simulink model "Histogram_equization_simulink"  (R2023b)
settings: Solver=VariableStepAuto  StartTime=0.0  StopTime=10.0  RelTol=1e-3
libraries: visionanalysis x1, visionsources x1
settings Model: Creator=snmz4  LastModifiedBy=snmz4

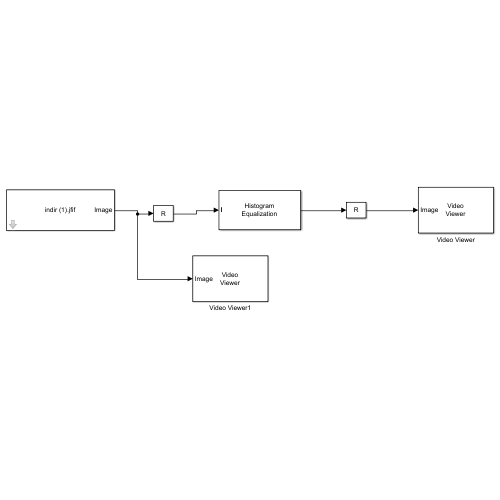
[thumbnail: Simulink's stored preview of the top-level diagram]
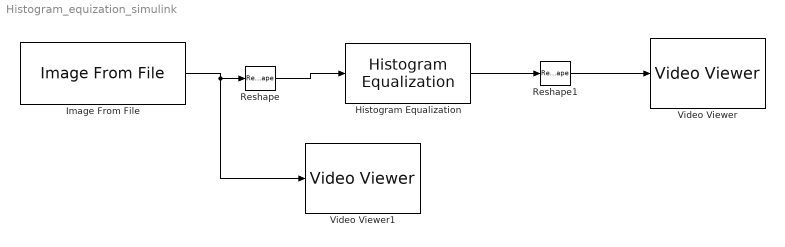
== system Histogram_equization_simulink ==
  Histogram Equalization : visionanalysis/Histogram Equalization  specify=Uniform  numbins=64  src=Specify via dialog  hist=ones(1,64)
  Image From File : visionsources/Image From File  Tag=vipblks_nd  FileName=C:\Users\snmz4\OneDrive\Resimler\indir (1).jfif  Ts=inf  imagePorts=One multidimensional signal  OutPortLabels=R|G|B  ImageDataType=double  sdImageDataType=uint(8)  Signed=on  WordLength=16  FractionLengthMode=User-defined  FractionLength=15
  Reshape : Reshape  OutputDimensionality=Customize  OutputDimensions=[225,225*3]
  Reshape1 : Reshape  OutputDimensionality=Customize  OutputDimensions=[225,225,3]
  Video Viewer : VideoViewer  FigPos=[719 521 418 304]
  Video Viewer1 : VideoViewer  FigPos=[279 522 418 304]
  wires:
  Image From File/1 -> Video Viewer1/1, Reshape/1
  Histogram Equalization/1 -> Reshape1/1
  Reshape/1 -> Histogram Equalization/1
  Reshape1/1 -> Video Viewer/1
